simulink model "hil_closed_loop_unified"  (R2026a)
settings: Solver=ode1  StopTime=inf  FixedStep=1/20
undefined symbols (not defined in the file or in its folder): read_cmdvel_live_interp, Sim3dSensor
libraries: sim3dcameralib x2, sim3dlib x1, uavsim3dlib x1
settings Model: SimulationMode=accelerator  Creator=Ahmed  LastModifiedBy=homie

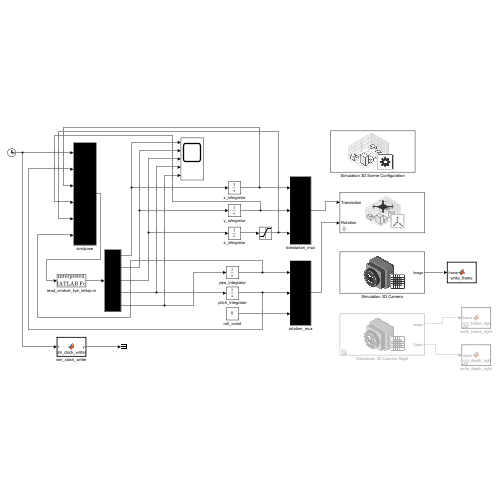
[thumbnail: Simulink's stored preview of the top-level diagram]
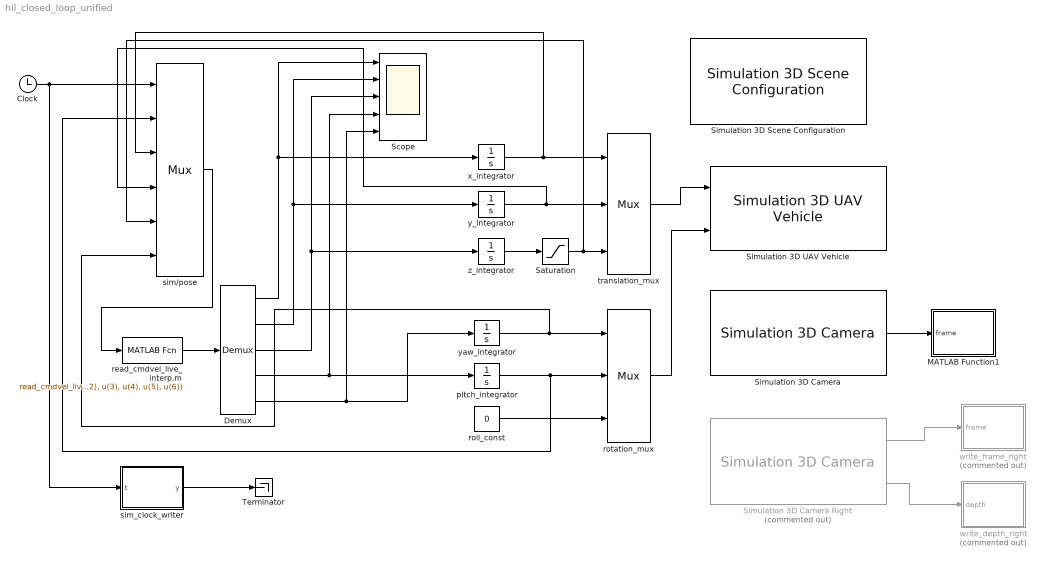
== system hil_closed_loop_unified ==
  Clock : Clock
  Demux : Demux  Outputs=5
  MATLAB Function1 : MATLAB Function  TreatAsAtomicUnit=on
  Saturation : Saturate  UpperLimit=80  LowerLimit=0
  Scope : Scope  NumInputPorts=5
      settings: ActiveDisplayYMinimum=-9.1502660334993  ActiveDisplayYMaximum=6.5758350892472208
  Simulation 3D Camera : sim3dcameralib/Simulation 3D Camera  Priority=1  sensorTag=Sim3dSensor�  sensorId=1  sensorName=Sim3dSensor�  vehTagList={'Custom ...';'Quadrotor1';'Scene Origin'}  vehTag=Quadrotor1  CoordinateSystem=ISO8855  mountLoc=Origin  offsetFlag=on  tmountOffset=[0.2, 0, 0.2]  extTmount=off  rmountOffset=[0, 5, 0]  extRmount=off  FocalLength=[554, 554]  OpticalCenter=[320, 240]  ImageSize=[480, 640]  RadialDistortion=[0, 0]  TangentialDistortion=[0, 0]  SensorSkew=0  VisualizeFieldOfView=off  FieldOfViewRange=61  DepthOutportEnabled=off  SemanticOutportEnabled=off  TransformOutportEnabled=off  SampleTime=-1  mountPoint=[0.2 0 0.2]  mountOrientation=[0 5 0]  aMode=4  ID=1
      settings: LibrarySourceBlock=uavsim3dlib/Simulation 3D Camera
  Simulation 3D Camera Right : sim3dcameralib/Simulation 3D Camera  Priority=1  Commented=on  sensorTag=Sim3dSensor�  sensorId=2  sensorName=Sim3dSensor�  vehTagList={'Custom ...';'Quadrotor1';'Scene Origin'}  vehTag=Quadrotor1  CoordinateSystem=ISO8855  mountLoc=Origin  offsetFlag=on  tmountOffset=[0.2, -0.11, 0.2]  extTmount=off  rmountOffset=[0, 5, 0]  extRmount=off  FocalLength=[554, 554]  OpticalCenter=[320, 240]  ImageSize=[480, 640]  RadialDistortion=[0, 0]  TangentialDistortion=[0, 0]  SensorSkew=0  VisualizeFieldOfView=off  FieldOfViewRange=61  DepthOutportEnabled=on  SemanticOutportEnabled=off  TransformOutportEnabled=off  SampleTime=-1  mountPoint=[0.2 -0.11 0.2]  mountOrientation=[0 5 0]  aMode=4  ID=2
      settings: LibrarySourceBlock=uavsim3dlib/Simulation 3D Camera
  Simulation 3D Scene Configuration : sim3dlib/Simulation 3D Scene Configuration  Priority=0  ProjectFormat=Default Scenes  SceneDesc=Large parking lot  ProjectName=C:\Program Files\MATLAB\R2026a\toolbox\shared\sim3d_projects\automotive_project_windows\UE\WindowsNoEditor\VehicleSimulation.exe  ScenePath=/Game/Maps/USCityBlock  EnableOpenDRIVE=off  vehTagList={'Custom';'Quadrotor1';'Scene Origin'}  vehTag=Quadrotor1  AttachedCameraRelativeTranslation=[0 0 0]  FreeCameraDefaultInitialTranslation=[-6, 0, 2]  AttachedCameraRelativeRotation=[0 0 0]  FreeCameraDefaultInitialRotation=[0, -15, 0]  ViewpointName=Custom  FreeCameraInitialTranslation=[0, 0, 0]  FreeCameraInitialRotation=[0, 0, 0]  OpVisEn=off  Ts=1/20  EnableWindow=on  EnableRemoteAccess=off  SimulationMode=CoSimulation  SimulateUsing=Interpreted execution  EnableAnimationRecording=off  OverrideDefaultRecording=off  AnimationRecordingFileName=sim3dAnimation.mat  AnimationRecordingInterval=[0 inf]  EnableWeather=off  SunAzimuth=90  SunAltitude=40.0  EnableGeospatialSun=off  Latitude=0  Longitude=0  Date=2023-01-01  Time=10:30:00  GeoTimeZone=-5.0  SunDaylightSaving=off  wind=1  clouds=10  EnableVolumetricClouds=off  CloudCoverage=0  CloudAltitude=6  fog=0  rain=0  RaindropsEffect=off  SnowDensity=0  EnableGeospatial=off  TilesetSource=Earth terrain  UseTrueOrigin=off  OriginHeight=200  OriginLatitude=40.744652  OriginLongitude=-73.988864  MapStyle=Aerial  AdditionalAssetIDs=[]  UseAdvancedSunSky=off  SolarTime=11  TimeZone=-5  Day=21  Month=9  Year=2022  UseDaylightSavingTime=on  DSTStartDay=10  DSTStartMonth=3  DSTEndDay=3  DSTEndMonth=11  DSTSwitchHour=2  sensorTag=MainCamera1  sensorId=1  sensorName=MainCamera1  mountLoc=Origin  offsetFlag=off  tmountOffset=[0, 0, 0]  rmountOffset=[0, 0, 0]  HorizontalResolution=1280  VerticalResolution=720  HorizontalFOV=60  mountPoint=[0 0 0]  mountOrientation=[0 0 0]  aMode=4  ID=1  GeoTrigger=Inactive  ViewNameList={'Custom'}  ViewTranslationList={'[0 0 0]'}  ViewRotationList={'[0 0 0]'}
      settings: LibrarySourceBlock=uavsim3dlib/Simulation 3D Scene Configuration
  Simulation 3D UAV Vehicle : uavsim3dlib/Simulation 3D UAV Vehicle  Priority=-1  Mesh=Quadrotor  MeshPath=/MathWorksUAVContent/UAVs/HexaRotorUAV/HexaRotor.HexaRotor  Color=Black  ActorName=Quadrotor1  UseGlobalFrame=off  InitialTranslation=[0 0 0]  InitialRotation=[0 0 0]  InitialTranslationGlobal=[0 0 0]  InitialGeoOrigin=[0 0 0]  InitialRotationGlobal=[0 0 0]  SampleTime=-1  ActorType=SimulinkVehicle  ID=C  aMode=4  ActorTag=Quadrotor1
  Terminator : Terminator
  pitch_integrator : Integrator
  read_cmdvel_live_interp.m : MATLABFcn  MATLABFcn=read_cmdvel_live_interp(u(1), u(2), u(3), u(4), u(5), u(6))
  roll_const : Constant  Value=0
  rotation_mux : Mux  Inputs=3
  sim/pose : Mux  Inputs=6
  sim_clock_writer : MATLAB Function  TreatAsAtomicUnit=on
  translation_mux : Mux  Inputs=3
  write_depth_right : MATLAB Function  Commented=on  TreatAsAtomicUnit=on
  write_frame_right : MATLAB Function  Commented=on  TreatAsAtomicUnit=on
  x_integrator : Integrator  InitialCondition=15.12
  y_integrator : Integrator  InitialCondition=3.84
  yaw_integrator : Integrator  InitialCondition=2*pi-0.0460
  z_integrator : Integrator  InitialCondition=7.5
  wires:
  Simulation 3D Camera/1 -> MATLAB Function1/1(frame)
  Demux/1 -> Scope/1, x_integrator/1
  Demux/2 -> Scope/2, y_integrator/1
  y_integrator/1 -> sim/pose/4, translation_mux/2
  translation_mux/1 -> Simulation 3D UAV Vehicle/1
  pitch_integrator/1 -> sim/pose/2, rotation_mux/2
  rotation_mux/1 -> Simulation 3D UAV Vehicle/2
  read_cmdvel_live_interp.m/1 -> Demux/1
  yaw_integrator/1 -> sim/pose/6, rotation_mux/1
  roll_const/1 -> rotation_mux/3
  Demux/3 -> Scope/3, z_integrator/1
  Saturation/1 -> sim/pose/5, translation_mux/3
  z_integrator/1 -> Saturation/1
  x_integrator/1 -> sim/pose/3, translation_mux/1
  Demux/4 -> Scope/4, pitch_integrator/1
  Demux/5 -> Scope/5, yaw_integrator/1
  Clock/1 -> sim_clock_writer/1(t), sim/pose/1
  sim/pose/1 -> read_cmdvel_live_interp.m/1
  sim_clock_writer/1(y) -> Terminator/1
  Simulation 3D Camera Right/1 -> write_frame_right/1(frame)
  Simulation 3D Camera Right/2 -> write_depth_right/1(depth)

== matlab function hil_closed_loop_unified/MATLAB Function1 ==
  data: frame input
function write_frame(frame)
coder.extrinsic('assignin');
assignin('base', 'latest_frame', frame);
end

== matlab function hil_closed_loop_unified/sim_clock_writer ==
  data: t input; y output
function y = sim_clock_writer(t)
%#codegen
% CRITICAL: this block must live inside Simulink, not in a MATLAB timer.
% It executes only when Simulink steps, so the Pi sees a frozen
% sim_heartbeat exactly when the simulator is paused / errored / hung.
    coder.extrinsic('assignin');
    assignin('base', 'sim_heartbeat', double(t));
    y = t;
end

== matlab function hil_closed_loop_unified/write_frame_right ==
  data: frame input
function write_frame_right(frame)
coder.extrinsic('assignin');
assignin('base', 'latest_frame_right', frame);
end

== matlab function hil_closed_loop_unified/write_depth_right ==
  data: depth input
function write_depth_right(depth)
coder.extrinsic('assignin');
assignin('base', 'latest_depth_right', depth);
end
